simulink library "flight_parameters_lib"  (R2018b)
settings: Solver=VariableStepAuto  StartTime=0.0  StopTime=10.0  RelTol=1e-3
settings Model: Creator=Ybeyer  LastModifiedBy=yannic
settings DebuggingCC: LibraryContextMissingDiagnostic=none
settings SFSimCC: SimUseLocalCustomCode=off
settings RTWCC: RTWUseLocalCustomCode=off
settings CodeAppCC: StateflowObjectComments=on

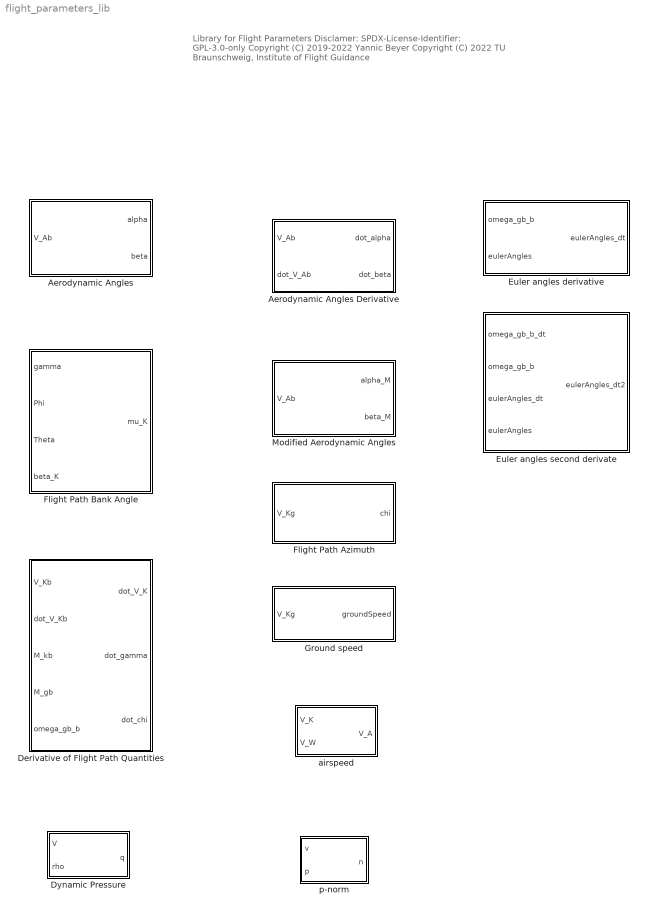
== system flight_parameters_lib ==
  note: Library for Flight Parameters
      |
      | Disclamer:
      | SPDX-License-Identifier: GPL-3.0-only
      |
      | Copyright (C) 2019-2022 Yannic Beyer
      | Copyright (C) 2022 TU Braunschweig, Institute of Flight Guidance
  Aerodynamic Angles : MATLAB Function  TreatAsAtomicUnit=on
  Aerodynamic Angles Derivative : MATLAB Function  TreatAsAtomicUnit=on
  Derivative of Flight Path Quantities : MATLAB Function  TreatAsAtomicUnit=on
  Dynamic Pressure : Subsystem
      mask DialogControl DescGroupVar Prompt: Compute the dynamic pressure from velocity and density
      mask DialogControl DescTextVar Prompt: q=1/2*rho*V^2
  Euler angles derivative : MATLAB Function  TreatAsAtomicUnit=on
  Euler angles second derivate : MATLAB Function  TreatAsAtomicUnit=on
  Flight Path Azimuth : MATLAB Function  TreatAsAtomicUnit=on
  "Flight Path Bank Angle " : MATLAB Function  TreatAsAtomicUnit=on
  Ground speed : MATLAB Function  TreatAsAtomicUnit=on
  Modified Aerodynamic Angles : MATLAB Function  TreatAsAtomicUnit=on
  airspeed : Subsystem
      mask DialogControl DescGroupVar Prompt: airspeed
      mask DialogControl DescTextVar Prompt: Compute airspeed from kinematic velocity and wind velocity
      mask DialogControl DescTextVar_copy Prompt: V_A = V_K - V_W
  p-norm : MATLAB Function  TreatAsAtomicUnit=on

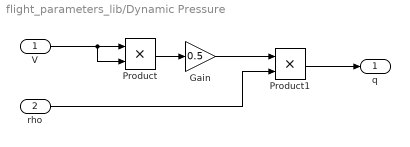
== system flight_parameters_lib/Dynamic Pressure ==
  V : Inport
  rho : Inport  Port=2
  Gain : Gain  Gain=0.5
  Product : Product
  Product1 : Product
  q : Outport
  wires:
  rho/1 -> Product1/2
  V/1 -> Product/2, Product/1
  Product1/1 -> q/1
  Product/1 -> Gain/1
  Gain/1 -> Product1/1

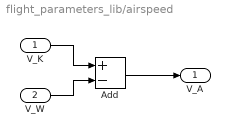
== system flight_parameters_lib/airspeed ==
  V_K : Inport
  V_W : Inport  Port=2
  Add : Sum  Inputs=+-
  V_A : Outport
  wires:
  V_W/1 -> Add/2
  Add/1 -> V_A/1
  V_K/1 -> Add/1

== matlab function flight_parameters_lib/Aerodynamic Angles Derivative ==
  data: V_Ab input; dot_alpha output; dot_V_Ab input; dot_beta output
function [ dot_alpha, dot_beta ] = fcn( V_Ab, dot_V_Ab ) %#codegen
[ dot_alpha, dot_beta ] = aeroAnglesDerivative( V_Ab, dot_V_Ab );

== matlab function flight_parameters_lib/Derivative of Flight Path Quantities ==
  data: V_Kb input; dot_V_K output; dot_V_Kb input; M_kb input; M_gb input; omega_gb_b input; dot_gamma output; dot_chi output
function [ dot_V_K, dot_gamma, dot_chi ] = fcn( ...
    V_Kb, dot_V_Kb, M_kb, M_gb, omega_gb_b ) %#codegen
[ dot_V_K, dot_gamma, dot_chi ] = flightPathDerivative( ...
    V_Kb, dot_V_Kb, M_kb, M_gb, omega_gb_b );

== matlab function flight_parameters_lib/p-norm ==
  data: v input; n output; p input
% norm computes the p-norm of a vector v 
%   https://de.mathworks.com/help/matlab/ref/norm.html
% *************************************************************************
function n = fcn(v,p) %#codegen
n = norm(v,p);

== matlab function flight_parameters_lib/Modified Aerodynamic Angles ==
  data: V_Ab input; alpha_M output; beta_M output
function [ alpha_M, beta_M ] = fcn( V_Ab ) %#codegen
[ alpha_M, beta_M ] = aeroAnglesMod( V_Ab );

== matlab function flight_parameters_lib/Flight Path Azimuth ==
  data: V_Kg input; chi output
function chi = fcn( V_Kg ) %#codegen
chi = flightPathAzimuth( V_Kg );
end

== matlab function flight_parameters_lib/Ground speed ==
  data: V_Kg input; groundSpeed output
% groundSpeed computes the absolute velocity of a point relative to 
%   the ground parallel to the horizontal plane.
% 
% Inputs:
%   V_Kg            flight path velocity represented in g frame (3xn vector
%                   where n is the number of flight path velocity vectors),
%                   in m/s
% 
% Outputs:
%   groundSpeed     ground speed (scalar or vector, depending on size
%                   of input), in m/s
% 
% See also: flightPathAzimuth
% 
%   Copyright 2019 TU Braunschweig
% *************************************************************************

function groundSpeed = groundSpeed( V_Kg ) %#codegen

% determine number of input vectors
num_vectors = length( V_Kg(1,:) );
groundSpeed = zeros( 1, num_vectors );
% compute the flight-path azimuth according to [1, page 58]
for i = 1:num_vectors
    groundSpeed(i) = norm( V_Kg(1:2,i), 2 );
end

end

== matlab function flight_parameters_lib/Euler angles derivative ==
  data: omega_gb_b input; eulerAngles_dt output; eulerAngles input
function eulerAngles_dt = fcn( omega_gb_b, eulerAngles ) %#codegen
    eulerAngles_dt = eulerDerivFromOmega( omega_gb_b, eulerAngles );
end

== matlab function flight_parameters_lib/Euler angles second derivate ==
  data: omega_gb_b_dt input; eulerAngles_dt2 output; omega_gb_b input; eulerAngles_dt input; eulerAngles input
function eulerAngles_dt2 = fcn( omega_gb_b_dt, ...
    omega_gb_b, eulerAngles_dt, eulerAngles ) %#codegen
    eulerAngles_dt2 = eulerDeriv2FromOmega( omega_gb_b_dt, ...
        omega_gb_b, eulerAngles_dt, eulerAngles );
end

== matlab function flight_parameters_lib/Aerodynamic Angles ==
  data: V_Ab input; alpha output; beta output
function [ alpha, beta ] = fcn( V_Ab ) %#codegen
[ alpha, beta ] = aeroAngles( V_Ab );

== matlab function flight_parameters_lib/Flight Path Bank Angle  ==
  data: gamma input; Phi input; Theta input; mu_K output; beta_K input
function mu_K = fcn( gamma, Phi, Theta, beta_K ) %#codegen
mu_K = flightPathBankAngle( gamma, Phi, Theta, beta_K );
